simulink model "A62_MPC_Sim"  (R2025b)
settings: Solver=FixedStepDiscrete  StartTime=0.0  StopTime=10  FixedStep=Tplant  RelTol=1e-3  EnableMultiTasking=on
values from neighbouring files (symbols this model uses):
  fr = 0.3    [CalcExp.m]    (also in Calculations.m)
  g = 9.81    [CalcExp.m]    (also in Calculations.m; workspace.mat)
  I = m*l^2/3    (= 0.0027225)    [CalcExp.m]    (also in Calculations.m; workspace.mat)
  K = lqr(A,B,Q,R)    [CalcExp.m]    (also in Calculations.m = lqr(A,B,diag([2000 0 1000 0]),R); rscale.m = k; workspace.mat = [-31.6227766017 -20.1449549457 72.7565036852 9.8125756249])
  l = 0.165    [CalcExp.m]    (also in Calculations.m; experiments.m = P.l*opt.lScale; workspace.mat)
  L = (place(A',C',EW))'    [CalcExp.m]    (also in Calculations.m; workspace.mat = [393.70593301  2.16234623159; 38748.8711552  425.852945691; )
  m = 0.3    [CalcExp.m]    (also in Calculations.m; experiments.m = runAll(makeCtl(c, P), SC, P, opt); workspace.mat)
  Nbar = rscale(sys_ss,K)    [CalcExp.m]    (also in Calculations.m; rscale.m = Nu + K*Nx; workspace.mat = -31.6227766017)
  nMPC = round(Ts*fISR)    [CalcExp.m]    (also in Calculations.m)
  spStepSize = 100    [CalcExp.m]    (also in Calculations.m)
  spStepTime = 3    [CalcExp.m]    (also in Calculations.m)
  theta0 = pi + 1.5*pi/180    (= 3.16777259237)    [CalcExp.m]    (also in Calculations.m)
  Tisr = 1/fISR    (= 0.002)    [CalcExp.m]    (also in Calculations.m; experiments.m = 1/ctl.fISR)
  Tplant = 1/8000    (= 0.000125)    [CalcExp.m]    (also in Calculations.m)
  useMPC = 1    [CalcExp.m]    (also in Calculations.m = double(startsWith(buildID, "M")))
  zRefD = LcD(:,1)'    [CalcExp.m]    (also in Calculations.m)
undefined symbols (not defined in the file or in its folder): DiscIntNeverNeededParam, mpcCore, mpcOnline, mpcState0
libraries: simulink x8, slpidlib x4
settings Model: ExtModeEnableFloating=off  Creator=The MathWorks, Inc.  LastModifiedBy=20100
settings SolverCC: AlgebraicLoopSolver=TrustRegion  AutoInsertRateTranBlk=on
settings DataIOCC: Decimation=8
settings OptimizationCC: DefaultParameterBehavior=Inlined  ExpressionDepthLimit=2147483647.0  InitFltsAndDblsToZero=on  MaxStackSize=64
settings DebuggingCC: UnderspecifiedInitializationDetection=Classic  MergeDetectMultiDrivingBlocksExec=none  CheckExecutionContextPreStartOutputMsg=on  SignalResolutionControl=TryResolveAllWithWarning  SolverPrmCheckMsg=warning  MultiTaskDSMMsg=warning  MultiTaskCondExecSysMsg=none  SigSpecEnsureSampleTimeMsg=none  FcnCallInpInsideContextMsg=warning  UnconnectedInputMsg=warning  UnconnectedOutputMsg=warning  UnconnectedLineMsg=warning  AllowSymbolicDim=off  StateNameClashWarn=warning  SFUnexpectedBacktrackingDiag=warning  SFNoUnconditionalDefaultTransitionDiag=warning  SFExecutionAtInitializationDiag=none  ArithmeticOperatorsInVariantConditions=warning
settings HardwareCC: ProdBitPerChar=16.0  ProdBitPerInt=16.0  ProdBitPerPointer=32.0  ProdLargestAtomicInteger=Integer  ProdLargestAtomicFloat=None  ProdWordSize=16.0  ProdHWDeviceType=Texas Instruments->C2000  TargetBitPerChar=16.0  TargetBitPerInt=16.0  TargetBitPerPointer=16.0  TargetLargestAtomicInteger=Integer  TargetIntDivRoundTo=Zero  TargetEndianess=LittleEndian  TargetWordSize=16.0  TargetHWDeviceType=Texas Instruments->C2000  ProdEqTarget=off
settings ModelReferenceCC: EnableRefExpFcnMdlSchedulingChecks=on  PropagateSignalLabelsOutOfModel=off
settings SFSimCC: SimUseLocalCustomCode=off  SimParseCustomCode=off  MATLABDynamicMemAlloc=off  CustomCodeUndefinedFunction=UseInterfaceOnly
settings RTWCC: PostCodeGenCommand=LNPostCodeGenCommand(modelName, buildInfo);  RTWUseLocalCustomCode=off  CustomInclude="\"C:\\Program Files\\LN\\MatlabToolbox\\lucasnuelle\\codelibs\""  GPUComputeCapability=3.5  DLArmComputeVersion=19.05
settings RTWCC: CustomSource=|
  | "C:\Program Files\LN\MatlabToolbox\lucasnuelle\codelibs\sfcn_lnc_wrapper.c"
  | "C:\Program Files\LN\MatlabToolbox\lucasnuelle\codelibs\CO36202A.c"
settings RTWCC: CustomLibrary=|
  | "C:\Program Files\LN\MatlabToolbox\lucasnuelle\codelibs\LNDacCO36202A.lib"
  | "C:\Program Files\LN\MatlabToolbox\lucasnuelle\codelibs\LNComCO36202A.lib"
  | "C:\Program Files\LN\MatlabToolbox\lucasnuelle\codelibs\LNDisplay.lib"
settings CodeAppCC: ForceParamTrailComments=on  StateflowObjectComments=on
settings GRTTargetCC: TargetLangStandard=C89/C90 (ANSI)
settings ConfigComp: CovSaveCumulativeToWorkspaceVar=on  CovSaveSingleToWorkspaceVar=on  CovExternalEMLEnable=off  CovSFcnEnable=off

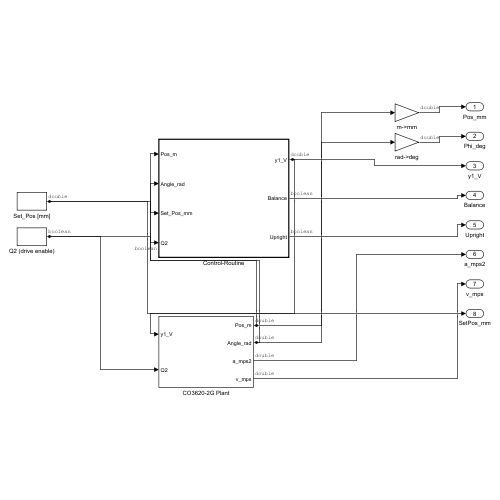
[thumbnail: Simulink's stored preview of the top-level diagram]
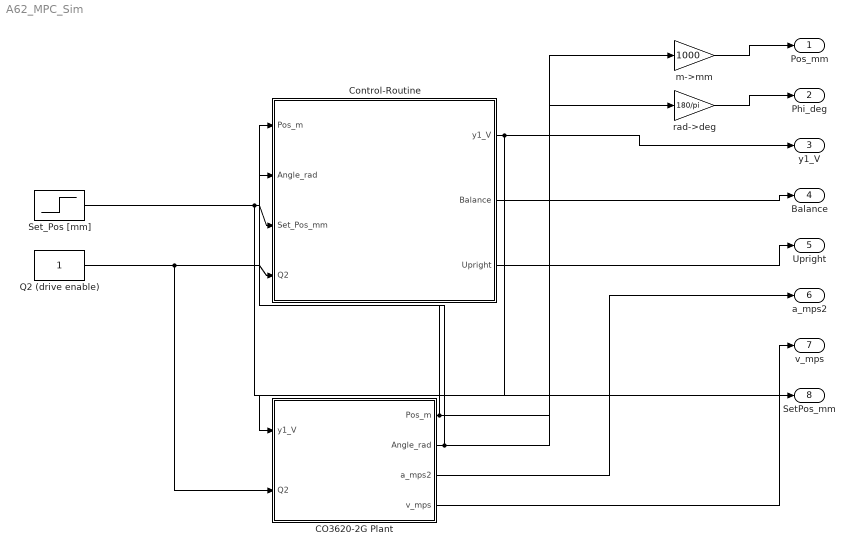
== system A62_MPC_Sim ==
  CO3620-2G Plant : Subsystem
  Control-Routine : Subsystem  TreatAsAtomicUnit=on  SystemSampleTime=Tisr  RTWFcnName=ControlInterruptSerivceRoutine
      settings: RTWSystemCode=Nonreusable function  RTWFcnNameOpts=User specified
  Q2 (drive enable) : Constant  OutDataTypeStr=boolean  SampleTime=Tisr
  Set_Pos [mm] : Step  Time=spStepTime  After=spStepSize  SampleTime=Tisr
  m->mm : Gain  Gain=1000
  rad->deg : Gain  Gain=180/pi
  Pos_mm : Outport
  Phi_deg : Outport  Port=2
  y1_V : Outport  Port=3
  Balance : Outport  Port=4
  Upright : Outport  Port=5
  a_mps2 : Outport  Port=6
  v_mps : Outport  Port=7
  SetPos_mm : Outport  Port=8
  wires:
  CO3620-2G Plant/1(Pos_m) -> Control-Routine/1(Pos_m), m->mm/1
  CO3620-2G Plant/2(Angle_rad) -> Control-Routine/2(Angle_rad), rad->deg/1
  Set_Pos [mm]/1 -> Control-Routine/3(Set_Pos_mm), SetPos_mm/1
  Q2 (drive enable)/1 -> Control-Routine/4(Q2), CO3620-2G Plant/2(Q2)
  Control-Routine/1(y1_V) -> CO3620-2G Plant/1(y1_V), y1_V/1
  m->mm/1 -> Pos_mm/1
  rad->deg/1 -> Phi_deg/1
  Control-Routine/2(Balance) -> Balance/1
  Control-Routine/3(Upright) -> Upright/1
  CO3620-2G Plant/3(a_mps2) -> a_mps2/1
  CO3620-2G Plant/4(v_mps) -> v_mps/1

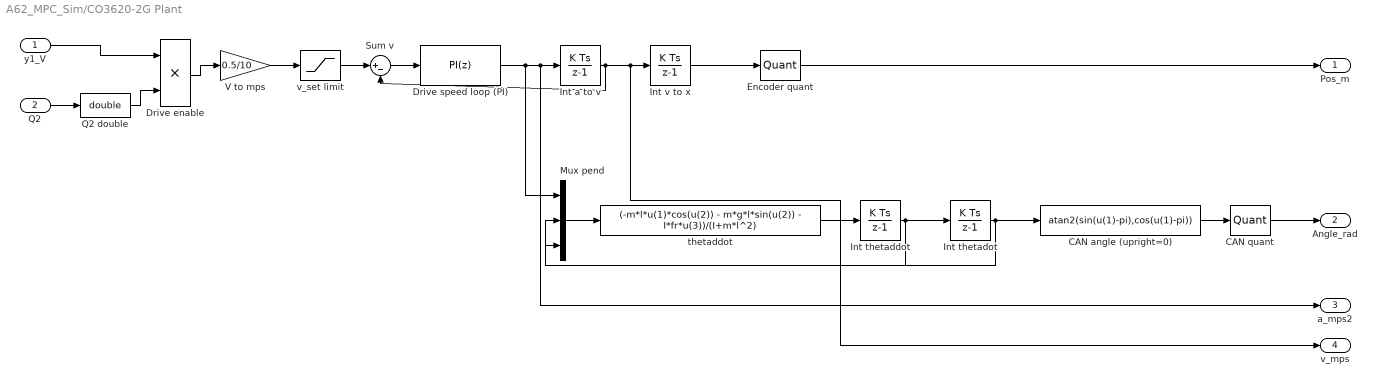
== system A62_MPC_Sim/CO3620-2G Plant ==
  y1_V : Inport
  Q2 : Inport  Port=2
  CAN angle (upright=0) : Fcn  Expr=atan2(sin(u(1)-pi),cos(u(1)-pi))
  CAN quant : Quantizer  QuantizationInterval=qAng
  Drive enable : Product
  Drive speed loop (PI) : slpidlib/PID Controller  Controller=PI  Form=Parallel  TimeDomain=Discrete-time  UseExternalTs=off  SampleTime=Tplant  IntegratorMethod=Forward Euler  FilterMethod=Forward Euler  ControllerParametersSource=internal  P=100  I=30  UseKiTs=off  D=0  UseExternalDerivativeSource=off  N=100  UseFilter=on  TunerSelectOption=Transfer Function Based (PID Tuner App)  InitialConditionSource=internal  InitialConditionForIntegrator=0  InitialConditionForFilter=0  DifferentiatorICPrevScaledInput=0  ExternalReset=none  TrackingMode=off  Kt=1  LimitOutput=on  SatLimitsSource=internal  UpperSaturationLimit=10  LowerSaturationLimit=-10  LinearizeAsGain=off  AntiWindupMode=back-calculation  Kb=1  LimitIntegrator=off  UpperIntegratorSaturationLimit=inf  LowerIntegratorSaturationLimit=-inf  POutMin=[]  POutMax=[]  IOutMin=[]  IOutMax=[]  DOutMin=[]  DOutMax=[]  NOutMin=[]  NOutMax=[]  SumOutMin=[]  SumOutMax=[]  SaturationOutMin=[]  SaturationOutMax=[]  PParamMin=[]  PParamMax=[]  IParamMin=[]  IParamMax=[]  DParamMin=[]  DParamMax=[]  NParamMin=[]  NParamMax=[]  KbParamMin=[]  KbParamMax=[]  KtParamMin=[]  KtParamMax=[]  KbOutMin=[]  KbOutMax=[]  KtOutMin=[]  KtOutMax=[]  IntegratorOutMin=[]  IntegratorOutMax=[]  FilterOutMin=[]  FilterOutMax=[]  SumI1OutMin=[]  SumI1OutMax=[]  SumI2OutMin=[]  SumI2OutMax=[]  SumI3OutMin=[]  SumI3OutMax=[]  SumI4OutMin=[]  SumI4OutMax=[]  SumDOutMin=[]  SumDOutMax=[]  DifferentiatorOutMin=[]  DifferentiatorOutMax=[]  FilterDiffOutCoefMin=[]  FilterDiffOutCoefMax=[]  ReciprocalOutMin=[]  ReciprocalOutMax=[]  SumDenOutMin=[]  SumDenOutMax=[]  SumNumOutMin=[]  SumNumOutMax=[]  DivideOutMin=[]  DivideOutMax=[]  UdiffTsProdOutMin=[]  UdiffTsProdOutMax=[]  NTsProdOutMin=[]  NTsProdOutMax=[]  UintegralTsProdOutMin=[]  UintegralTsProdOutMax=[]  UngainTsProdOutMin=[]  UngainTsProdOutMax=[]  ClampingZeroOutDataTypeStr=Inherit: Inherit via back propagation  ClampingZeroOutMin=[]  ClampingZeroOutMax=[]  FilterDenConstantOutDataTypeStr=Inherit: Inherit via back propagation  FilterDenConstantOutMin=[]  FilterDenConstantOutMax=[]  PCopyOutDataTypeStr=Inherit: Inherit via back propagation  PCopyOutMin=[]  PCopyOutMax=[]  NCopyOutDataTypeStr=Inherit: Inherit via back propagation  NCopyOutMin=[]  NCopyOutMax=[]  IntegratorContinuousStateAttributes=''  IntegratorStateMustResolveToSignalObject=off  IntegratorRTWStateStorageClass=Auto  FilterContinuousStateAttributes=''  FilterStateMustResolveToSignalObject=off  FilterRTWStateStorageClass=Auto  ParallelPVariant=InternalParameters  IdealPVariant=Disabled  IVariant=InternalParameters  DVariant=Disabled  IntegratorVariant=Discrete  SatVariant=Enabled  AWVariant=BackCalculation  PCopyVariant=Disabled  TRVariant=Disabled  FdbkBlocksVariant=Forward  IdealPFdbkVariant=Disabled  SatFdbkVariant=Disabled  DerivativeFilterVariant=Disabled  NVariant=Disabled  NCopyVariant=Disabled_SignalSpec  FilterICVariant=Disabled  IntegratorICVariant=InternalICs  ExternalResetVariant=Disabled  TRSumVariant=Passthrough  SumFdbkVariant=Disabled  SumVariant=Sum_PI  TsampFilterVariant=InternalTs  TsampNgainVariant=Passthrough  TsampIntegralVariant=Disabled_SignalSpec  ExternalSaturationOutDataTypeStr=Inherit: Same as second input  DerivativeSourceVariant=Disabled  PreIntVariant=InternalPreInt
      settings: LibrarySourceBlock=simulink/Discrete/Discrete PID Controller
  Encoder quant : Quantizer  QuantizationInterval=qPos
  Int a to v : DiscreteIntegrator  SampleTime=Tplant  ICPrevOutput=DiscIntNeverNeededParam  ICPrevScaledInput=DiscIntNeverNeededParam
  Int thetaddot : DiscreteIntegrator  SampleTime=Tplant  ICPrevOutput=DiscIntNeverNeededParam  ICPrevScaledInput=DiscIntNeverNeededParam
  Int thetadot : DiscreteIntegrator  InitialCondition=theta0  SampleTime=Tplant  ICPrevOutput=DiscIntNeverNeededParam  ICPrevScaledInput=DiscIntNeverNeededParam
  Int v to x : DiscreteIntegrator  SampleTime=Tplant  ICPrevOutput=DiscIntNeverNeededParam  ICPrevScaledInput=DiscIntNeverNeededParam
  Mux pend : Mux  Inputs=3
  Q2 double : DataTypeConversion  OutDataTypeStr=double  SaturateOnIntegerOverflow=off  RndMeth=Floor
  Sum v : Sum  Inputs=|+-
  V to mps : Gain  Gain=0.5/10
  thetaddot : Fcn  Expr=(-m*l*u(1)*cos(u(2)) - m*g*l*sin(u(2)) - I*fr*u(3))/(I+m*l^2)
  v_set limit : Saturate
  Pos_m : Outport
  Angle_rad : Outport  Port=2
  a_mps2 : Outport  Port=3
  v_mps : Outport  Port=4
  wires:
  Q2/1 -> Q2 double/1
  y1_V/1 -> Drive enable/1
  Q2 double/1 -> Drive enable/2
  Drive enable/1 -> V to mps/1
  V to mps/1 -> v_set limit/1
  v_set limit/1 -> Sum v/1
  Sum v/1 -> Drive speed loop (PI)/1
  Drive speed loop (PI)/1 -> Int a to v/1, a_mps2/1, Mux pend/1
  Int a to v/1 -> Int v to x/1, v_mps/1, Sum v/2
  Int v to x/1 -> Encoder quant/1
  Encoder quant/1 -> Pos_m/1
  Int thetadot/1 -> Mux pend/2, CAN angle (upright=0)/1
  Int thetaddot/1 -> Mux pend/3, Int thetadot/1
  Mux pend/1 -> thetaddot/1
  thetaddot/1 -> Int thetaddot/1
  CAN angle (upright=0)/1 -> CAN quant/1
  CAN quant/1 -> Angle_rad/1

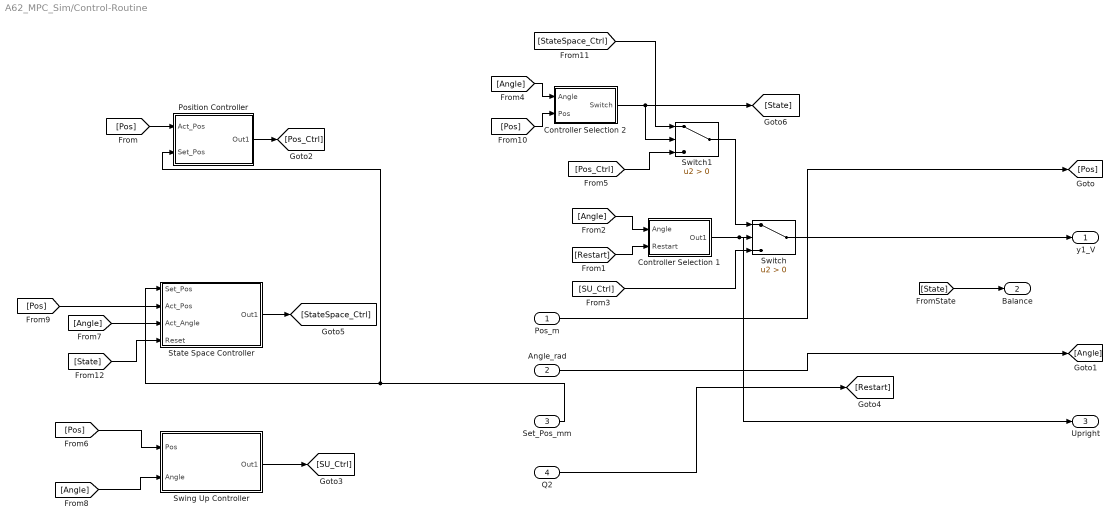
== system A62_MPC_Sim/Control-Routine ==
  Pos_m : Inport
  Angle_rad : Inport  Port=2
  Set_Pos_mm : Inport  Port=3
  Q2 : Inport  Port=4  OutDataTypeStr=boolean
  Controller Selection 1 : Subsystem
  Controller Selection 2 : Subsystem
  Position Controller : Subsystem
  State Space Controller : Subsystem
  Swing Up Controller : Subsystem
  Switch : Switch  Criteria=u2 > Threshold  SaturateOnIntegerOverflow=off  InputSameDT=off
  Switch1 : Switch  Criteria=u2 > Threshold  SaturateOnIntegerOverflow=off  InputSameDT=off
  y1_V : Outport
  Balance : Outport  Port=2
  Upright : Outport  Port=3
  wires:
  [StateSpace_Ctrl] -> Switch1/1
  [Pos] -> Controller Selection 2/2(Pos)
  [Angle] -> Controller Selection 2/1(Angle)
  Controller Selection 2/1(Switch) -> [State], Switch1/2
  [Pos_Ctrl] -> Switch1/3
  Switch1/1 -> Switch/1
  [State] -> State Space Controller/4(Reset)
  [Restart] -> Controller Selection 1/2(Restart)
  Swing Up Controller/1(Out1) -> [SU_Ctrl]
  [Angle] -> Swing Up Controller/2(Angle)
  [Pos] -> Swing Up Controller/1(Pos)
  [Pos] -> State Space Controller/2(Act_Pos)
  [Angle] -> State Space Controller/3(Act_Angle)
  State Space Controller/1(Out1) -> [StateSpace_Ctrl]
  [SU_Ctrl] -> Switch/3
  [Angle] -> Controller Selection 1/1(Angle)
  Controller Selection 1/1(Out1) -> Switch/2, Upright/1
  Position Controller/1(Out1) -> [Pos_Ctrl]
  [Pos] -> Position Controller/1(Act_Pos)
  Pos_m/1 -> [Pos]
  Angle_rad/1 -> [Angle]
  Set_Pos_mm/1 -> Position Controller/2(Set_Pos), State Space Controller/1(Set_Pos)
  Q2/1 -> [Restart]
  Switch/1 -> y1_V/1
  [State] -> Balance/1

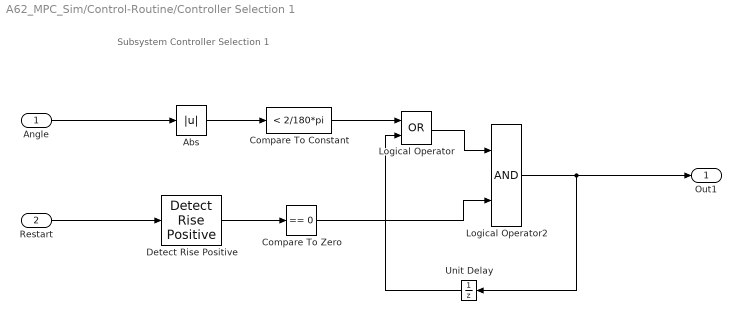
== system A62_MPC_Sim/Control-Routine/Controller Selection 1 ==
  note: Subsystem Controller Selection 1
  Angle : Inport
  Restart : Inport  Port=2
  Abs : Abs  SaturateOnIntegerOverflow=off
  Compare To Constant : simulink/Logic and Bit Operations/Compare To Constant  relop=<  const=2/180*pi  OutDataTypeStr=boolean
  Compare To Zero : simulink/Logic and Bit Operations/Compare To Zero  relop===  OutDataTypeStr=boolean
  Detect Rise Positive : simulink/Logic and Bit Operations/Detect Rise Positive  vinit=0  OutDataTypeStr=boolean
  Logical Operator : Logic  Operator=OR  AllPortsSameDT=off  OutDataTypeStr=boolean
  Logical Operator2 : Logic  AllPortsSameDT=off  OutDataTypeStr=boolean
  Unit Delay : UnitDelay  SampleTime=-1  HasFrameUpgradeWarning=on
  Out1 : Outport
  wires:
  Unit Delay/1 -> Logical Operator/2
  Angle/1 -> Abs/1
  Abs/1 -> Compare To Constant/1
  Logical Operator/1 -> Logical Operator2/1
  Compare To Constant/1 -> Logical Operator/1
  Logical Operator2/1 -> Unit Delay/1, Out1/1
  Restart/1 -> Detect Rise Positive/1
  Detect Rise Positive/1 -> Compare To Zero/1
  Compare To Zero/1 -> Logical Operator2/2

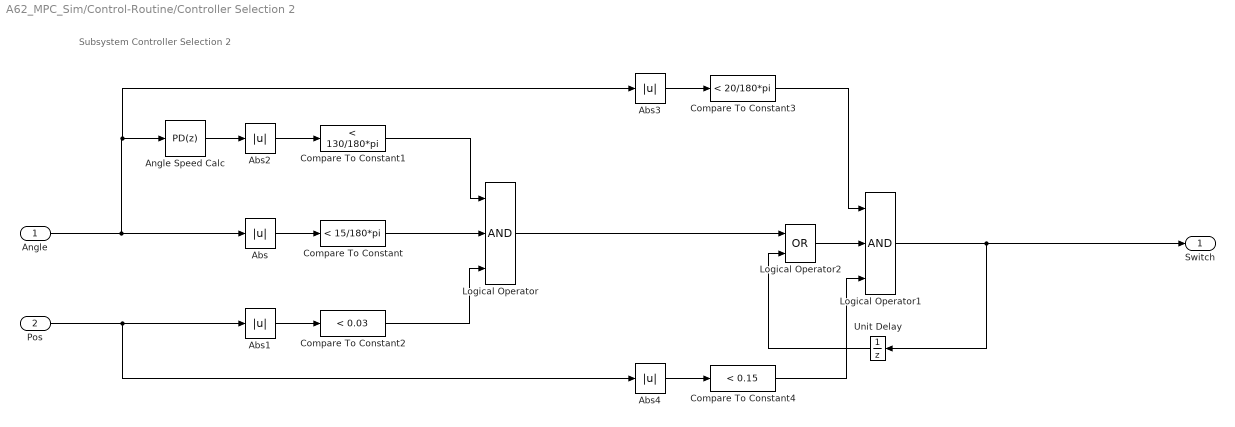
== system A62_MPC_Sim/Control-Routine/Controller Selection 2 ==
  note: Subsystem Controller Selection 2
  Angle : Inport
  Pos : Inport  Port=2
  Abs{,1..4} (5 alike) : Abs  SaturateOnIntegerOverflow=off
  Angle Speed Calc : slpidlib/PID Controller  Controller=PD  Form=Parallel  TimeDomain=Discrete-time  UseExternalTs=off  SampleTime=-1  IntegratorMethod=Forward Euler  FilterMethod=Forward Euler  ControllerParametersSource=internal  P=0  I=1  UseKiTs=off  D=1  UseExternalDerivativeSource=off  N=100  UseFilter=on  TunerSelectOption=Transfer Function Based (PID Tuner App)  InitialConditionSource=internal  InitialConditionForIntegrator=0  InitialConditionForFilter=0  DifferentiatorICPrevScaledInput=0  ExternalReset=none  TrackingMode=off  Kt=1  LimitOutput=off  SatLimitsSource=internal  UpperSaturationLimit=inf  LowerSaturationLimit=-inf  LinearizeAsGain=off  AntiWindupMode=none  Kb=1  LimitIntegrator=off  UpperIntegratorSaturationLimit=inf  LowerIntegratorSaturationLimit=-inf  POutMin=[]  POutMax=[]  IOutMin=[]  IOutMax=[]  DOutMin=[]  DOutMax=[]  NOutMin=[]  NOutMax=[]  SumOutMin=[]  SumOutMax=[]  SaturationOutMin=[]  SaturationOutMax=[]  PParamMin=[]  PParamMax=[]  IParamMin=[]  IParamMax=[]  DParamMin=[]  DParamMax=[]  NParamMin=[]  NParamMax=[]  KbParamMin=[]  KbParamMax=[]  KtParamMin=[]  KtParamMax=[]  KbOutMin=[]  KbOutMax=[]  KtOutMin=[]  KtOutMax=[]  IntegratorOutMin=[]  IntegratorOutMax=[]  FilterOutMin=[]  FilterOutMax=[]  SumI1OutMin=[]  SumI1OutMax=[]  SumI2OutMin=[]  SumI2OutMax=[]  SumI3OutMin=[]  SumI3OutMax=[]  SumI4OutMin=[]  SumI4OutMax=[]  SumDOutMin=[]  SumDOutMax=[]  DifferentiatorOutMin=[]  DifferentiatorOutMax=[]  FilterDiffOutCoefMin=[]  FilterDiffOutCoefMax=[]  ReciprocalOutMin=[]  ReciprocalOutMax=[]  SumDenOutMin=[]  SumDenOutMax=[]  SumNumOutMin=[]  SumNumOutMax=[]  DivideOutMin=[]  DivideOutMax=[]  UdiffTsProdOutMin=[]  UdiffTsProdOutMax=[]  NTsProdOutMin=[]  NTsProdOutMax=[]  UintegralTsProdOutMin=[]  UintegralTsProdOutMax=[]  UngainTsProdOutMin=[]  UngainTsProdOutMax=[]  ClampingZeroOutDataTypeStr=Inherit: Inherit via back propagation  ClampingZeroOutMin=[]  ClampingZeroOutMax=[]  FilterDenConstantOutDataTypeStr=Inherit: Inherit via back propagation  FilterDenConstantOutMin=[]  FilterDenConstantOutMax=[]  PCopyOutDataTypeStr=Inherit: Inherit via back propagation  PCopyOutMin=[]  PCopyOutMax=[]  NCopyOutDataTypeStr=Inherit: Inherit via back propagation  NCopyOutMin=[]  NCopyOutMax=[]  IntegratorContinuousStateAttributes=''  IntegratorStateMustResolveToSignalObject=off  IntegratorRTWStateStorageClass=Auto  FilterContinuousStateAttributes=''  FilterStateMustResolveToSignalObject=off  FilterRTWStateStorageClass=Auto  ParallelPVariant=InternalParameters  IdealPVariant=Disabled  IVariant=Disabled  DVariant=InternalParameters  IntegratorVariant=Disabled  SatVariant=Disabled  AWVariant=Disabled  PCopyVariant=Disabled  TRVariant=Disabled  FdbkBlocksVariant=Forward  IdealPFdbkVariant=Disabled  SatFdbkVariant=Disabled  DerivativeFilterVariant=ForwardEulerFilter  NVariant=InternalParameters  NCopyVariant=Disabled  FilterICVariant=InternalICsFilter  IntegratorICVariant=Disabled  ExternalResetVariant=Disabled  TRSumVariant=Passthrough  SumFdbkVariant=Disabled  SumVariant=Sum_PD  TsampFilterVariant=InternalTs  TsampNgainVariant=Passthrough  TsampIntegralVariant=Disabled_SignalSpec  ExternalSaturationOutDataTypeStr=Inherit: Same as second input  DerivativeSourceVariant=ErrorSignal  PreIntVariant=InternalPreInt
  Compare To Constant : simulink/Logic and Bit Operations/Compare To Constant  relop=<  const=15/180*pi  OutDataTypeStr=boolean
  Compare To Constant1 : simulink/Logic and Bit Operations/Compare To Constant  relop=<  const=130/180*pi  OutDataTypeStr=boolean
  Compare To Constant2 : simulink/Logic and Bit Operations/Compare To Constant  relop=<  const=0.03  OutDataTypeStr=boolean
  Compare To Constant3 : simulink/Logic and Bit Operations/Compare To Constant  relop=<  const=20/180*pi  OutDataTypeStr=boolean
  Compare To Constant4 : simulink/Logic and Bit Operations/Compare To Constant  relop=<  const=0.15  OutDataTypeStr=boolean
  Logical Operator : Logic  Inputs=3  AllPortsSameDT=off  OutDataTypeStr=boolean
  Logical Operator1 : Logic  Inputs=3  AllPortsSameDT=off  OutDataTypeStr=boolean
  Logical Operator2 : Logic  Operator=OR  AllPortsSameDT=off  OutDataTypeStr=boolean
  Unit Delay : UnitDelay  SampleTime=-1  HasFrameUpgradeWarning=on
  Switch : Outport
  wires:
  Logical Operator/1 -> Logical Operator2/1
  Abs/1 -> Compare To Constant/1
  Angle/1 -> Abs/1, Abs3/1, Angle Speed Calc/1
  Abs1/1 -> Compare To Constant2/1
  Compare To Constant/1 -> Logical Operator/2
  Pos/1 -> Abs4/1, Abs1/1
  Compare To Constant2/1 -> Logical Operator/3
  Logical Operator2/1 -> Logical Operator1/2
  Logical Operator1/1 -> Unit Delay/1, Switch/1
  Unit Delay/1 -> Logical Operator2/2
  Abs2/1 -> Compare To Constant1/1
  Compare To Constant1/1 -> Logical Operator/1
  Angle Speed Calc/1 -> Abs2/1
  Abs3/1 -> Compare To Constant3/1
  Compare To Constant3/1 -> Logical Operator1/1
  Abs4/1 -> Compare To Constant4/1
  Compare To Constant4/1 -> Logical Operator1/3

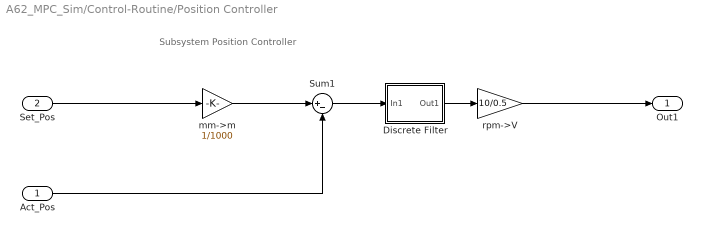
== system A62_MPC_Sim/Control-Routine/Position Controller ==
  note: Subsystem Position Controller
  Act_Pos : Inport
  Set_Pos : Inport  Port=2
  Discrete Filter : Subsystem
  Sum1 : Sum  Inputs=|+-
  mm->m : Gain  Gain=1/1000
  rpm->V : Gain  Gain=10/0.5
  Out1 : Outport
  wires:
  rpm->V/1 -> Out1/1
  Set_Pos/1 -> mm->m/1
  Discrete Filter/1(Out1) -> rpm->V/1
  Sum1/1 -> Discrete Filter/1(In1)
  mm->m/1 -> Sum1/1
  Act_Pos/1 -> Sum1/2

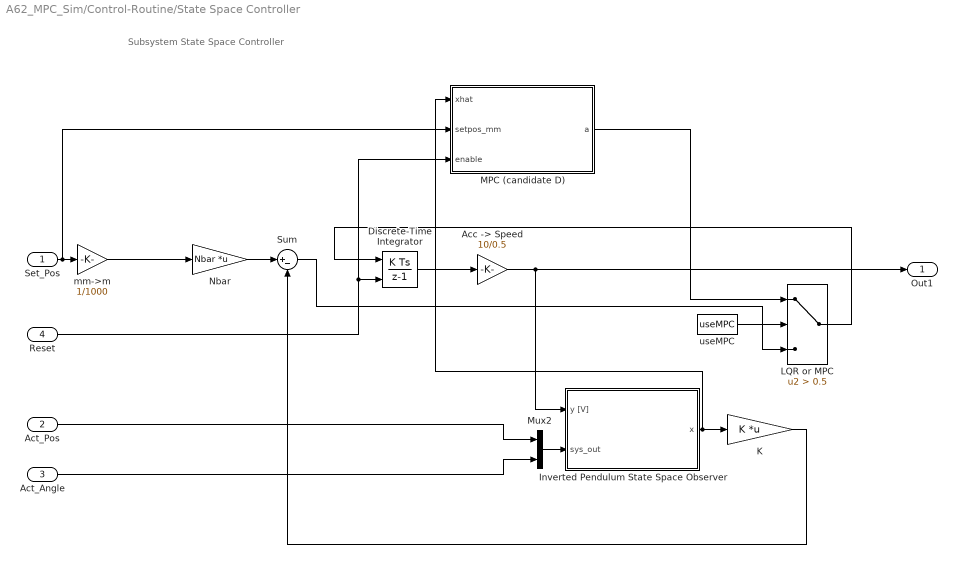
== system A62_MPC_Sim/Control-Routine/State Space Controller ==
  note: Subsystem State Space Controller
  Set_Pos : Inport
  Act_Pos : Inport  Port=2
  Act_Angle : Inport  Port=3
  Reset : Inport  Port=4
  "Acc -> Speed" : Gain  Gain=10/0.5
  Discrete-Time Integrator : DiscreteIntegrator  ExternalReset=rising  SampleTime=-1  ICPrevOutput=DiscIntNeverNeededParam  ICPrevScaledInput=DiscIntNeverNeededParam
  Inverted Pendulum State Space Observer : Subsystem  mask{DefSystem=Predefined, b=[], m=0.3, l=0.165, fr=0.3, exportData=on}
      mask prompts: DefSystem "Predefined System"; b "coefficient of friction for cart"; m "mass of the pendulum [kg]"; l "length to pendulum center of mass [m]"; fr "pendulum friction"; exportData "Export System Parameter"
      mask init:
      | I = m*l^2/3;
      | g = 9.81;
      | 
      | A=[ 0 1 0 0;
      |     0 0 0 0
      |     0 0 0 1
      |     0 0 m*g*l/(I+m*l^2) 0];
      | B=[0;1;0;m*l/(I+m*l^2)];
      | C=[ 1 0 0 0
      |     0 0 1 0];
      | 
      | % Export parameter to matlab workspace
      | if ((strcmpi(get_param(gcb, 'exportData'), 'on')))
      |     assignin('base', 'A', A);
      |     assignin('base', 'B', B);
      |     assignin('base', 'C', C);
      | end
      mask TypeOptions DefSystem: Predefined | User defined
      mask Callback DefSystem:
      | fu = LNInvertedPendulumSystemWrapper();
      | fu.ParamFcn(gcb);
      mask Display:
      | color('white');
      | plot([0 20],[0 20]);
      | 
      | color('orange');
      | port_label('input', 1, 'y [V]');
      | port_label('input', 2, 'sys_out');
      | port_label('output', 1, 'x');
      | 
      | color('orange');
      | text(8,18, 'LN-Sim');
  K : Gain  Gain=K  Multiplication=Matrix(K*u) (u vector)
  LQR or MPC : Switch  Criteria=u2 > Threshold  Threshold=0.5  SaturateOnIntegerOverflow=off  InputSameDT=off
  MPC (candidate D) : MATLAB Function  TreatAsAtomicUnit=on
  Mux2 : Mux  Inputs=2
  Nbar : Gain  Gain=Nbar  Multiplication=Matrix(K*u) (u vector)
  Sum : Sum  Inputs=|+-
  mm->m : Gain  Gain=1/1000
  useMPC : Constant  Value=useMPC
  Out1 : Outport
  wires:
  "Acc -> Speed"/1 -> Out1/1, Inverted Pendulum State Space Observer/1(y [V])
  K/1 -> Sum/2
  Act_Pos/1 -> Mux2/1
  Mux2/1 -> Inverted Pendulum State Space Observer/2(sys_out)
  Act_Angle/1 -> Mux2/2
  Nbar/1 -> Sum/1
  Inverted Pendulum State Space Observer/1(x) -> K/1, MPC (candidate D)/1(xhat)
  Discrete-Time Integrator/1 -> "Acc -> Speed"/1
  Set_Pos/1 -> mm->m/1, MPC (candidate D)/2(setpos_mm)
  Reset/1 -> Discrete-Time Integrator/2, MPC (candidate D)/3(enable)
  mm->m/1 -> Nbar/1
  MPC (candidate D)/1(a) -> LQR or MPC/1
  useMPC/1 -> LQR or MPC/2
  Sum/1 -> LQR or MPC/3
  LQR or MPC/1 -> Discrete-Time Integrator/1

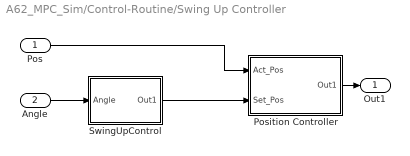
== system A62_MPC_Sim/Control-Routine/Swing Up Controller ==
  Pos : Inport
  Angle : Inport  Port=2
  Position Controller : Subsystem
  SwingUpControl : Subsystem
  Out1 : Outport
  wires:
  Pos/1 -> Position Controller/1(Act_Pos)
  SwingUpControl/1(Out1) -> Position Controller/2(Set_Pos)
  Position Controller/1(Out1) -> Out1/1
  Angle/1 -> SwingUpControl/1(Angle)

== system A62_MPC_Sim/Control-Routine/Position Controller/Discrete Filter ==
  note: Subsystem Discrete PT1
  In1 : Inport
  Discrete-Time Integrator : DiscreteIntegrator  gainval=1/0.17  SampleTime=-1  ICPrevOutput=DiscIntNeverNeededParam  ICPrevScaledInput=DiscIntNeverNeededParam
  K : Gain  Gain=4.17
  Sum1 : Sum  Inputs=|+-
  Out1 : Outport
  wires:
  Sum1/1 -> Discrete-Time Integrator/1
  In1/1 -> K/1
  K/1 -> Sum1/1
  Discrete-Time Integrator/1 -> Out1/1, Sum1/2

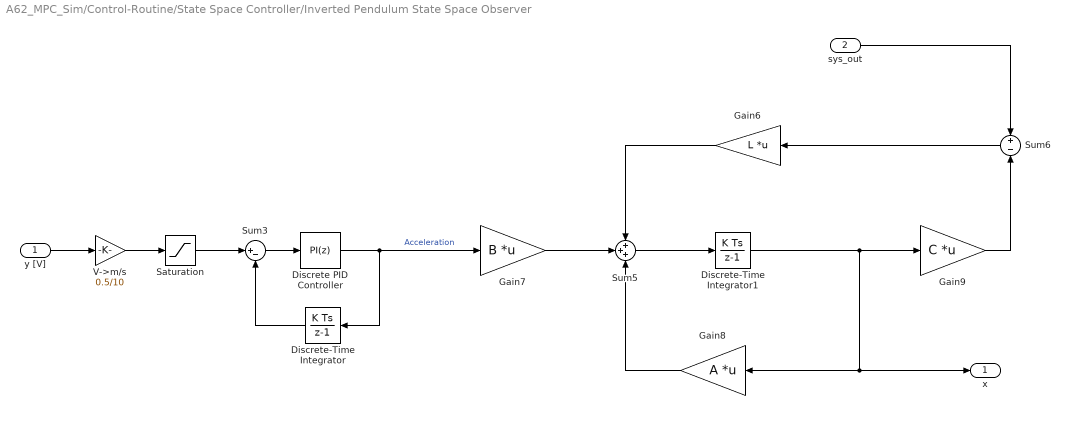
== system A62_MPC_Sim/Control-Routine/State Space Controller/Inverted Pendulum State Space Observer ==
  y [V] : Inport
  sys_out : Inport  Port=2
  Discrete PID Controller : slpidlib/PID Controller  Controller=PI  Form=Parallel  TimeDomain=Discrete-time  UseExternalTs=off  SampleTime=-1  IntegratorMethod=Forward Euler  FilterMethod=Forward Euler  ControllerParametersSource=internal  P=100  I=30  UseKiTs=off  D=0  UseExternalDerivativeSource=off  N=100  UseFilter=on  TunerSelectOption=Transfer Function Based (PID Tuner App)  InitialConditionSource=internal  InitialConditionForIntegrator=0  InitialConditionForFilter=0  DifferentiatorICPrevScaledInput=0  ExternalReset=none  TrackingMode=off  Kt=1  LimitOutput=on  SatLimitsSource=internal  UpperSaturationLimit=10  LowerSaturationLimit=-10  LinearizeAsGain=off  AntiWindupMode=back-calculation  Kb=1  LimitIntegrator=off  UpperIntegratorSaturationLimit=inf  LowerIntegratorSaturationLimit=-inf  POutMin=[]  POutMax=[]  IOutMin=[]  IOutMax=[]  DOutMin=[]  DOutMax=[]  NOutMin=[]  NOutMax=[]  SumOutMin=[]  SumOutMax=[]  SaturationOutMin=[]  SaturationOutMax=[]  PParamMin=[]  PParamMax=[]  IParamMin=[]  IParamMax=[]  DParamMin=[]  DParamMax=[]  NParamMin=[]  NParamMax=[]  KbParamMin=[]  KbParamMax=[]  KtParamMin=[]  KtParamMax=[]  KbOutMin=[]  KbOutMax=[]  KtOutMin=[]  KtOutMax=[]  IntegratorOutMin=[]  IntegratorOutMax=[]  FilterOutMin=[]  FilterOutMax=[]  SumI1OutMin=[]  SumI1OutMax=[]  SumI2OutMin=[]  SumI2OutMax=[]  SumI3OutMin=[]  SumI3OutMax=[]  SumI4OutMin=[]  SumI4OutMax=[]  SumDOutMin=[]  SumDOutMax=[]  DifferentiatorOutMin=[]  DifferentiatorOutMax=[]  FilterDiffOutCoefMin=[]  FilterDiffOutCoefMax=[]  ReciprocalOutMin=[]  ReciprocalOutMax=[]  SumDenOutMin=[]  SumDenOutMax=[]  SumNumOutMin=[]  SumNumOutMax=[]  DivideOutMin=[]  DivideOutMax=[]  UdiffTsProdOutMin=[]  UdiffTsProdOutMax=[]  NTsProdOutMin=[]  NTsProdOutMax=[]  UintegralTsProdOutMin=[]  UintegralTsProdOutMax=[]  UngainTsProdOutMin=[]  UngainTsProdOutMax=[]  ClampingZeroOutDataTypeStr=Inherit: Inherit via back propagation  ClampingZeroOutMin=[]  ClampingZeroOutMax=[]  FilterDenConstantOutDataTypeStr=Inherit: Inherit via back propagation  FilterDenConstantOutMin=[]  FilterDenConstantOutMax=[]  PCopyOutDataTypeStr=Inherit: Inherit via back propagation  PCopyOutMin=[]  PCopyOutMax=[]  NCopyOutDataTypeStr=Inherit: Inherit via back propagation  NCopyOutMin=[]  NCopyOutMax=[]  IntegratorContinuousStateAttributes=''  IntegratorStateMustResolveToSignalObject=off  IntegratorRTWStateStorageClass=Auto  FilterContinuousStateAttributes=''  FilterStateMustResolveToSignalObject=off  FilterRTWStateStorageClass=Auto  ParallelPVariant=InternalParameters  IdealPVariant=Disabled  IVariant=InternalParameters  DVariant=Disabled  IntegratorVariant=Discrete  SatVariant=Enabled  AWVariant=BackCalculation  PCopyVariant=Disabled  TRVariant=Disabled  FdbkBlocksVariant=Forward  IdealPFdbkVariant=Disabled  SatFdbkVariant=Disabled  DerivativeFilterVariant=Disabled  NVariant=Disabled  NCopyVariant=Disabled_SignalSpec  FilterICVariant=Disabled  IntegratorICVariant=InternalICs  ExternalResetVariant=Disabled  TRSumVariant=Passthrough  SumFdbkVariant=Disabled  SumVariant=Sum_PI  TsampFilterVariant=InternalTs  TsampNgainVariant=Passthrough  TsampIntegralVariant=Disabled_SignalSpec  ExternalSaturationOutDataTypeStr=Inherit: Same as second input  DerivativeSourceVariant=Disabled  PreIntVariant=InternalPreInt
  Discrete-Time Integrator : DiscreteIntegrator  SampleTime=-1  ICPrevOutput=DiscIntNeverNeededParam  ICPrevScaledInput=DiscIntNeverNeededParam
  Discrete-Time Integrator1 : DiscreteIntegrator  SampleTime=-1  ICPrevOutput=DiscIntNeverNeededParam  ICPrevScaledInput=DiscIntNeverNeededParam
  Gain6 : Gain  Gain=L  Multiplication=Matrix(K*u) (u vector)
  Gain7 : Gain  Gain=B  Multiplication=Matrix(K*u) (u vector)
  Gain8 : Gain  Gain=A  Multiplication=Matrix(K*u) (u vector)
  Gain9 : Gain  Gain=C  Multiplication=Matrix(K*u) (u vector)
  Saturation : Saturate
  Sum3 : Sum  Inputs=|+-
  Sum5 : Sum  Inputs=+++
  Sum6 : Sum  Inputs=+|-
  V->m/s : Gain  Gain=0.5/10
  x : Outport
  wires:
  sys_out/1 -> Sum6/1
  Gain8/1 -> Sum5/3
  Sum6/1 -> Gain6/1
  Discrete-Time Integrator1/1 -> x/1, Gain8/1, Gain9/1
  Discrete-Time Integrator/1 -> Sum3/2
  Gain9/1 -> Sum6/2
  V->m/s/1 -> Saturation/1
  y [V]/1 -> V->m/s/1
  Discrete PID Controller/1 -> Discrete-Time Integrator/1, Gain7/1  "Acceleration"
  Gain6/1 -> Sum5/1
  Sum3/1 -> Discrete PID Controller/1
  Gain7/1 -> Sum5/2
  Sum5/1 -> Discrete-Time Integrator1/1
  Saturation/1 -> Sum3/1

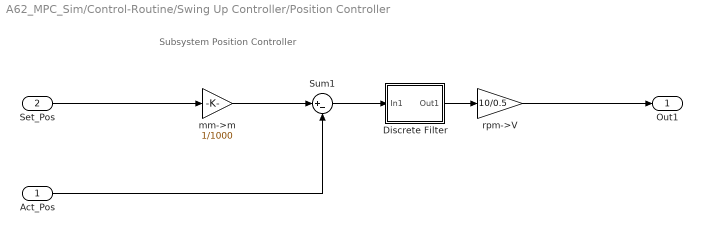
== system A62_MPC_Sim/Control-Routine/Swing Up Controller/Position Controller ==
  note: Subsystem Position Controller
  Act_Pos : Inport
  Set_Pos : Inport  Port=2
  Discrete Filter : Subsystem
  Sum1 : Sum  Inputs=|+-
  mm->m : Gain  Gain=1/1000
  rpm->V : Gain  Gain=10/0.5
  Out1 : Outport
  wires:
  rpm->V/1 -> Out1/1
  Set_Pos/1 -> mm->m/1
  Discrete Filter/1(Out1) -> rpm->V/1
  Sum1/1 -> Discrete Filter/1(In1)
  mm->m/1 -> Sum1/1
  Act_Pos/1 -> Sum1/2

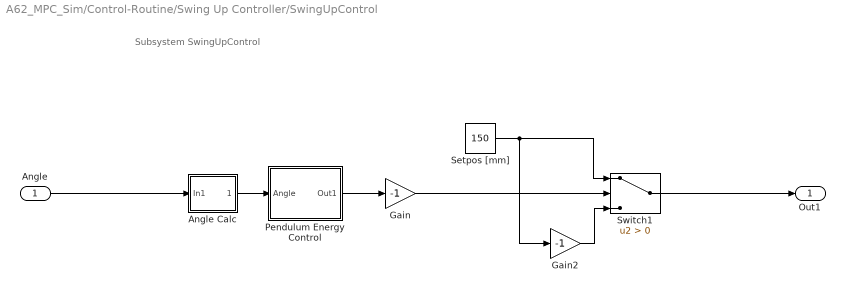
== system A62_MPC_Sim/Control-Routine/Swing Up Controller/SwingUpControl ==
  note: Subsystem SwingUpControl
  Angle : Inport
  Angle Calc : Subsystem
  Gain : Gain  Gain=-1
  Gain2 : Gain  Gain=-1
  Pendulum Energy Control : Subsystem
  Setpos [mm] : Constant  Value=150
  Switch1 : Switch  Criteria=u2 > Threshold  SaturateOnIntegerOverflow=off  InputSameDT=off
  Out1 : Outport
  wires:
  Setpos [mm]/1 -> Gain2/1, Switch1/1
  Gain/1 -> Switch1/2
  Angle/1 -> Angle Calc/1(In1)
  Switch1/1 -> Out1/1
  Pendulum Energy Control/1(Out1) -> Gain/1
  Gain2/1 -> Switch1/3
  Angle Calc/1(Out1) -> Pendulum Energy Control/1(Angle)

== system A62_MPC_Sim/Control-Routine/Swing Up Controller/Position Controller/Discrete Filter ==
  note: Subsystem Discrete PT1
  In1 : Inport
  Discrete-Time Integrator : DiscreteIntegrator  gainval=1/0.17  SampleTime=-1  ICPrevOutput=DiscIntNeverNeededParam  ICPrevScaledInput=DiscIntNeverNeededParam
  K : Gain  Gain=4.17
  Sum1 : Sum  Inputs=|+-
  Out1 : Outport
  wires:
  Sum1/1 -> Discrete-Time Integrator/1
  In1/1 -> K/1
  K/1 -> Sum1/1
  Discrete-Time Integrator/1 -> Out1/1, Sum1/2

== system A62_MPC_Sim/Control-Routine/Swing Up Controller/SwingUpControl/Angle Calc ==
  note: Subsystem Angle Calc
  In1 : Inport
  Constant : Constant  Value=-2*pi
  Sum : Sum  Inputs=|++
  Switch : Switch  Criteria=u2 > Threshold  SaturateOnIntegerOverflow=off  InputSameDT=off
  Out1 : Outport
  wires:
  Sum/1 -> Switch/1
  Constant/1 -> Sum/1
  In1/1 -> Switch/2, Sum/2, Switch/3
  Switch/1 -> Out1/1

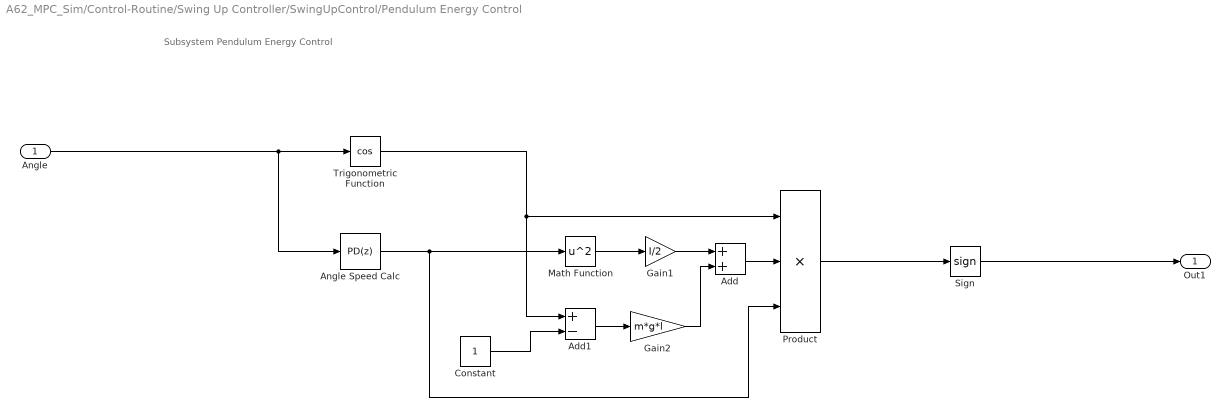
== system A62_MPC_Sim/Control-Routine/Swing Up Controller/SwingUpControl/Pendulum Energy Control ==
  note: Subsystem Pendulum Energy Control
  Angle : Inport
  Add : Sum
  Add1 : Sum  Inputs=+-
  Angle Speed Calc : slpidlib/PID Controller  Controller=PD  Form=Parallel  TimeDomain=Discrete-time  UseExternalTs=off  SampleTime=-1  IntegratorMethod=Forward Euler  FilterMethod=Forward Euler  ControllerParametersSource=internal  P=0  I=1  UseKiTs=off  D=1  UseExternalDerivativeSource=off  N=100  UseFilter=on  TunerSelectOption=Transfer Function Based (PID Tuner App)  InitialConditionSource=internal  InitialConditionForIntegrator=0  InitialConditionForFilter=0  DifferentiatorICPrevScaledInput=0  ExternalReset=none  TrackingMode=off  Kt=1  LimitOutput=off  SatLimitsSource=internal  UpperSaturationLimit=inf  LowerSaturationLimit=-inf  LinearizeAsGain=off  AntiWindupMode=none  Kb=1  LimitIntegrator=off  UpperIntegratorSaturationLimit=inf  LowerIntegratorSaturationLimit=-inf  POutMin=[]  POutMax=[]  IOutMin=[]  IOutMax=[]  DOutMin=[]  DOutMax=[]  NOutMin=[]  NOutMax=[]  SumOutMin=[]  SumOutMax=[]  SaturationOutMin=[]  SaturationOutMax=[]  PParamMin=[]  PParamMax=[]  IParamMin=[]  IParamMax=[]  DParamMin=[]  DParamMax=[]  NParamMin=[]  NParamMax=[]  KbParamMin=[]  KbParamMax=[]  KtParamMin=[]  KtParamMax=[]  KbOutMin=[]  KbOutMax=[]  KtOutMin=[]  KtOutMax=[]  IntegratorOutMin=[]  IntegratorOutMax=[]  FilterOutMin=[]  FilterOutMax=[]  SumI1OutMin=[]  SumI1OutMax=[]  SumI2OutMin=[]  SumI2OutMax=[]  SumI3OutMin=[]  SumI3OutMax=[]  SumI4OutMin=[]  SumI4OutMax=[]  SumDOutMin=[]  SumDOutMax=[]  DifferentiatorOutMin=[]  DifferentiatorOutMax=[]  FilterDiffOutCoefMin=[]  FilterDiffOutCoefMax=[]  ReciprocalOutMin=[]  ReciprocalOutMax=[]  SumDenOutMin=[]  SumDenOutMax=[]  SumNumOutMin=[]  SumNumOutMax=[]  DivideOutMin=[]  DivideOutMax=[]  UdiffTsProdOutMin=[]  UdiffTsProdOutMax=[]  NTsProdOutMin=[]  NTsProdOutMax=[]  UintegralTsProdOutMin=[]  UintegralTsProdOutMax=[]  UngainTsProdOutMin=[]  UngainTsProdOutMax=[]  ClampingZeroOutDataTypeStr=Inherit: Inherit via back propagation  ClampingZeroOutMin=[]  ClampingZeroOutMax=[]  FilterDenConstantOutDataTypeStr=Inherit: Inherit via back propagation  FilterDenConstantOutMin=[]  FilterDenConstantOutMax=[]  PCopyOutDataTypeStr=Inherit: Inherit via back propagation  PCopyOutMin=[]  PCopyOutMax=[]  NCopyOutDataTypeStr=Inherit: Inherit via back propagation  NCopyOutMin=[]  NCopyOutMax=[]  IntegratorContinuousStateAttributes=''  IntegratorStateMustResolveToSignalObject=off  IntegratorRTWStateStorageClass=Auto  FilterContinuousStateAttributes=''  FilterStateMustResolveToSignalObject=off  FilterRTWStateStorageClass=Auto  ParallelPVariant=InternalParameters  IdealPVariant=Disabled  IVariant=Disabled  DVariant=InternalParameters  IntegratorVariant=Disabled  SatVariant=Disabled  AWVariant=Disabled  PCopyVariant=Disabled  TRVariant=Disabled  FdbkBlocksVariant=Forward  IdealPFdbkVariant=Disabled  SatFdbkVariant=Disabled  DerivativeFilterVariant=ForwardEulerFilter  NVariant=InternalParameters  NCopyVariant=Disabled  FilterICVariant=InternalICsFilter  IntegratorICVariant=Disabled  ExternalResetVariant=Disabled  TRSumVariant=Passthrough  SumFdbkVariant=Disabled  SumVariant=Sum_PD  TsampFilterVariant=InternalTs  TsampNgainVariant=Passthrough  TsampIntegralVariant=Disabled_SignalSpec  ExternalSaturationOutDataTypeStr=Inherit: Same as second input  DerivativeSourceVariant=ErrorSignal  PreIntVariant=InternalPreInt
  Constant : Constant  SampleTime=-1
  Gain1 : Gain  Gain=I/2
  Gain2 : Gain  Gain=m*g*l
  Math Function : Math  Operator=square  SignedPower=on
  Product : Product  Inputs=3
  Sign : Signum
  Trigonometric Function : Trigonometry  Operator=cos
  Out1 : Outport
  wires:
  Math Function/1 -> Gain1/1
  Angle/1 -> Trigonometric Function/1, Angle Speed Calc/1
  Constant/1 -> Add1/2
  Gain2/1 -> Add/2
  Add1/1 -> Gain2/1
  Gain1/1 -> Add/1
  Add/1 -> Product/2
  Sign/1 -> Out1/1
  Product/1 -> Sign/1
  Angle Speed Calc/1 -> Math Function/1, Product/3
  Trigonometric Function/1 -> Product/1, Add1/1

== matlab function A62_MPC_Sim/Control-Routine/State Space Controller/MPC (candidate D) ==
  data: xhat input; a output; setpos_mm input; enable input; mpcCore parameter; mpcState0 parameter; mpcOnline parameter; zRefD parameter; nMPC parameter
function a = MPC_D(xhat, setpos_mm, enable, mpcCore, mpcState0, mpcOnline, zRefD, nMPC)
%#codegen
% MPC (candidate D) called every nMPC-th Control-Routine call (100 Hz).
% xhat = [x; xdot; phi; phidot] from the LN state observer (custom state estimate).
% Computed in SINGLE precision: on the F28335 (TI C28x, COFF) double is only 32 bit.
persistent sd cnt aHold
if isempty(sd)
    sd = mpcState0;  cnt = 0;  aHold = single(0);
end
if enable
    if cnt == 0
        r  = single(setpos_mm)/single(1000);           % set-point [m]
        od = mpcOnline;
        od.signals.ym  = single([xhat(1); xhat(3)]);   % measured outputs x, phi
        od.signals.ref = [r single(0) single(0) r*single(zRefD)];   % [x phi xdot z1..z4]
        sd.Plant = single(xhat(:));                    % custom state estimation
        [aHold, sd] = mpcmoveCodeGeneration(mpcCore, sd, od);
    end
    cnt = cnt + 1;
    if cnt >= nMPC
        cnt = 0;
    end
else
    cnt = 0;  aHold = single(0);  sd = mpcState0;      % not balancing: reset
end
a = double(aHold);
